simulink model "ex5_3"  (R2026a)
settings: Solver=FixedStepAuto  StopTime=2  FixedStep=0.001
settings Model: Creator=User  LastModifiedBy=User

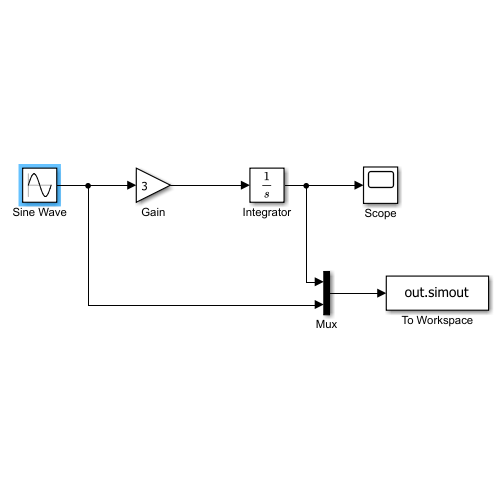
[thumbnail: Simulink's stored preview of the top-level diagram]
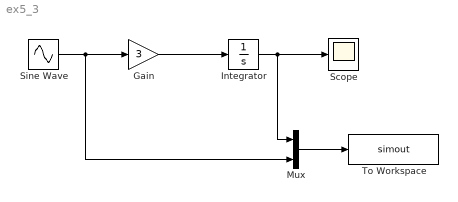
== system ex5_3 ==
  Gain : Gain  Gain=3
  Integrator : Integrator
  Mux : Mux  Inputs=2
  Scope : Scope
  Sine Wave : Sin  Frequency=2*pi  SampleTime=0
  To Workspace : ToWorkspace  VariableName=simout  SaveFormat=Timeseries  SampleTime=-1
  wires:
  Sine Wave/1 -> Mux/2, Gain/1
  Gain/1 -> Integrator/1
  Integrator/1 -> Scope/1, Mux/1
  Mux/1 -> To Workspace/1
